simulink model "EV_BMS_SOC_Estimation_System"  (R2026a)
settings: Solver=ode4  StopTime=SCN.t_end  FixedStep=0.25
values from neighbouring files (symbols this model uses):
  BMS = struct('I_dis_cont', 20, 'I_chg_cont', 4,      'T_warn', 45, 'T_derate', 50, 'T_cutoff', 60,      'T_chg_min', 0, 'T_chg_low', 10, 'T_chg_max', 50,      'T_cold', -20, 'V_max', 4.20, 'V_min', 2.80, 'SOC_min', 0.05,      'enable', g('bms_enable', 1))    [ev_scenario.m]
  ET = struct()    [ET_Battery_Params.m]    (also in run_Extreme_Heat_Scenarios.m = apply_cooling(ET0, S{k,7}); run_Indian_Climate_Scenarios.m = apply_cooling(ET0, S{k,6}))
  PACK = struct('Ns', 20, 'Np', 14)    [ev_scenario.m]
  SCN = struct()    [ev_scenario.m]
  VEH = struct('name', 'Electric scooter', 'm', 195,              'Cd', 0.70, 'A', 0.85, 'Crr', 0.016, 'rho', 1.18, 'kr', 1.03,              'eta_drive', 0.85, 'eta_regen', 0.50, 'P_regen_max', 2e3,              'P_trac_max', 6e3, 'v_regen_min', 5)    [ev_scenario.m]
libraries: sl_discontinuities x1
settings Model: Creator=anand  LastModifiedBy=anand

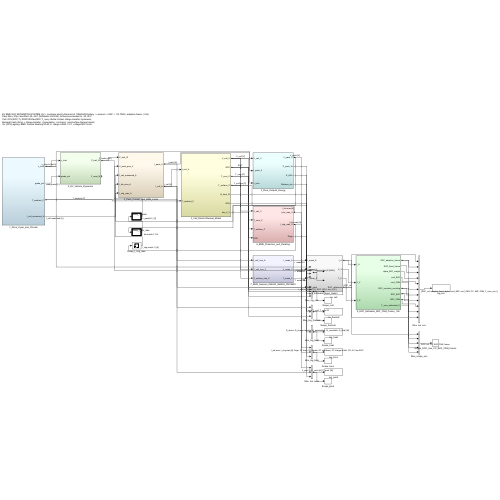
[thumbnail: Simulink's stored preview of the top-level diagram]
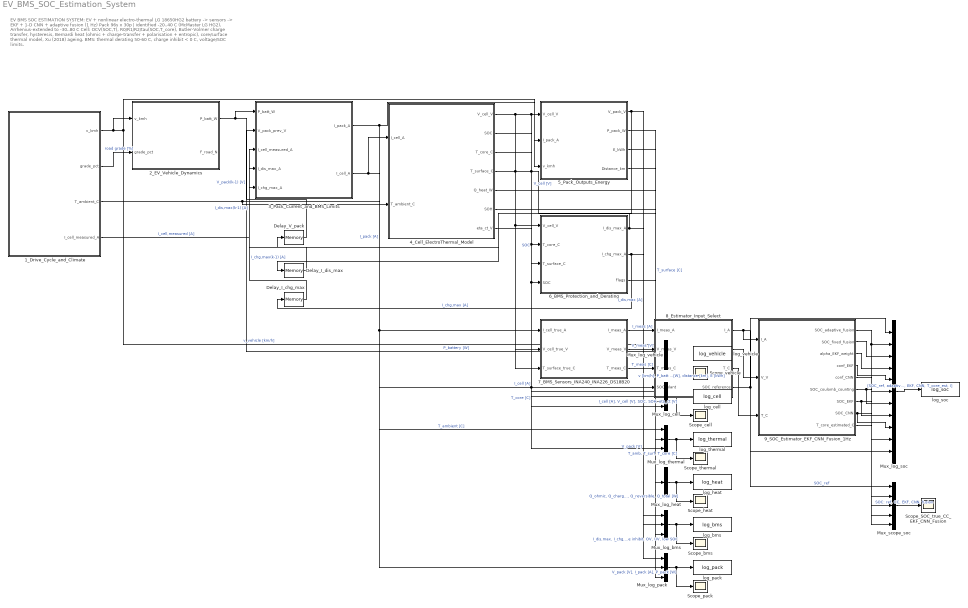
== system EV_BMS_SOC_Estimation_System ==
  note: EV BMS SOC ESTIMATION SYSTEM: EV + nonlinear electro-thermal LG 18650HG2 battery -> sensors -> EKF + 1-D CNN + adaptive fusion (1 Hz)
      | Pack 96s x 30p | identified -20..40 C (McMaster LG HG2), Arrhenius-extended to -30..80 C
      | Cell: OCV(SOC,T), R0/R1/R2/tau(SOC,T_core), Butler-Volmer charge transfer, hysteresis,
      | Bernardi heat (ohmic + charge-transfer + polarisation + entropic), core/surface thermal model,
      | Xu (2018) ageing. BMS: thermal derating 50-60 C, charge inhibit < 0 C, voltage/SOC limits.
  1_Drive_Cycle_and_Climate : Subsystem
  2_EV_Vehicle_Dynamics : Subsystem
  3_Pack_Current_and_BMS_Limits : Subsystem
  4_Cell_ElectroThermal_Model : Subsystem
  5_Pack_Outputs_Energy : Subsystem
  6_BMS_Protection_and_Derating : Subsystem
  7_BMS_Sensors_INA240_INA226_DS18B20 : Subsystem
  8_Estimator_Input_Select : Subsystem
  9_SOC_Estimator_EKF_CNN_Fusion_1Hz : Subsystem
  Delay_I_chg_max : Memory  InitialCondition=BMS.I_chg_cont*PACK.Np
  Delay_I_dis_max : Memory  InitialCondition=BMS.I_dis_cont*PACK.Np
  Delay_V_pack : Memory  InitialCondition=PACK.Ns*3.7
  Mux_log_bms : Mux  Inputs=3
  Mux_log_cell : Mux  Inputs=5
  Mux_log_heat : Mux  Inputs=1
  Mux_log_pack : Mux  Inputs=3
  Mux_log_soc : Mux  Inputs=11
  Mux_log_thermal : Mux  Inputs=3
  Mux_log_vehicle : Mux
  Mux_scope_soc : Mux  Inputs=5
  Scope_SOC_true_CC_EKF_CNN_Fusion : Scope
  Scope_bms : Scope
  Scope_cell : Scope
  Scope_heat : Scope
  Scope_pack : Scope
  Scope_thermal : Scope
  Scope_vehicle : Scope
  log_bms : ToWorkspace  VariableName=log_bms  SaveFormat=Timeseries  SampleTime=-1
  log_cell : ToWorkspace  VariableName=log_cell  SaveFormat=Timeseries  SampleTime=-1
  log_heat : ToWorkspace  VariableName=log_heat  SaveFormat=Timeseries  SampleTime=-1
  log_pack : ToWorkspace  VariableName=log_pack  SaveFormat=Timeseries  SampleTime=-1
  log_soc : ToWorkspace  VariableName=log_soc  SaveFormat=Timeseries  SampleTime=-1
  log_thermal : ToWorkspace  VariableName=log_thermal  SaveFormat=Timeseries  SampleTime=-1
  log_vehicle : ToWorkspace  VariableName=log_vehicle  SaveFormat=Timeseries  SampleTime=-1
  wires:
  1_Drive_Cycle_and_Climate/1(v_kmh) -> 5_Pack_Outputs_Energy/3(v_kmh), Mux_log_vehicle/1, 2_EV_Vehicle_Dynamics/1(v_kmh)  "v_vehicle [km/h]"
  1_Drive_Cycle_and_Climate/2(grade_pct) -> 2_EV_Vehicle_Dynamics/2(grade_pct)  "road grade [%]"
  1_Drive_Cycle_and_Climate/3(T_ambient_C) -> 4_Cell_ElectroThermal_Model/2(T_ambient_C), Mux_log_thermal/1  "T_ambient [C]"
  1_Drive_Cycle_and_Climate/4(I_cell_measured_A) -> 3_Pack_Current_and_BMS_Limits/3(I_cell_measured_A)  "I_cell,measured [A]"
  2_EV_Vehicle_Dynamics/1(P_batt_W) -> 3_Pack_Current_and_BMS_Limits/1(P_batt_W), Mux_log_vehicle/2  "P_battery [W]"
  Delay_V_pack/1 -> 3_Pack_Current_and_BMS_Limits/2(V_pack_prev_V)  "V_pack(k-1) [V]"
  Delay_I_dis_max/1 -> 3_Pack_Current_and_BMS_Limits/4(I_dis_max_A)  "I_dis,max(k-1) [A]"
  Delay_I_chg_max/1 -> 3_Pack_Current_and_BMS_Limits/5(I_chg_max_A)  "I_chg,max(k-1) [A]"
  3_Pack_Current_and_BMS_Limits/2(I_cell_A) -> Mux_log_cell/1, 7_BMS_Sensors_INA240_INA226_DS18B20/1(I_cell_true_A), 4_Cell_ElectroThermal_Model/1(I_cell_A)  "I_cell [A]"
  3_Pack_Current_and_BMS_Limits/1(I_pack_A) -> 5_Pack_Outputs_Energy/2(I_pack_A), Mux_log_pack/2  "I_pack [A]"
  4_Cell_ElectroThermal_Model/1(V_cell_V) -> 6_BMS_Protection_and_Derating/1(V_cell_V), 7_BMS_Sensors_INA240_INA226_DS18B20/2(V_cell_true_V), 5_Pack_Outputs_Energy/1(V_cell_V), Mux_log_cell/2  "V_cell [V]"
  5_Pack_Outputs_Energy/1(V_pack_V) -> Delay_V_pack/1, Mux_log_pack/1  "V_pack [V]"
  4_Cell_ElectroThermal_Model/3(T_core_C) -> 6_BMS_Protection_and_Derating/2(T_core_C), Mux_log_thermal/3  "T_core [C]"
  4_Cell_ElectroThermal_Model/4(T_surface_C) -> 6_BMS_Protection_and_Derating/3(T_surface_C), Mux_log_thermal/2, 7_BMS_Sensors_INA240_INA226_DS18B20/3(T_surface_true_C)  "T_surface [C]"
  4_Cell_ElectroThermal_Model/2(SOC) -> Mux_log_cell/3, 8_Estimator_Input_Select/4(SOC_plant), 6_BMS_Protection_and_Derating/4(SOC)  "SOC"
  6_BMS_Protection_and_Derating/1(I_dis_max_A) -> Delay_I_dis_max/1, Mux_log_bms/1  "I_dis,max [A]"
  6_BMS_Protection_and_Derating/2(I_chg_max_A) -> Delay_I_chg_max/1, Mux_log_bms/2  "I_chg,max [A]"
  5_Pack_Outputs_Energy/4(Distance_km) -> Mux_log_vehicle/3
  5_Pack_Outputs_Energy/3(E_kWh) -> Mux_log_vehicle/4
  Mux_log_vehicle/1 -> log_vehicle/1, Scope_vehicle/1  "v [km/h], P_batt [W], distance [km], E [kWh]"
  4_Cell_ElectroThermal_Model/6(SOH) -> Mux_log_cell/4
  4_Cell_ElectroThermal_Model/7(eta_ct_V) -> Mux_log_cell/5
  Mux_log_cell/1 -> log_cell/1, Scope_cell/1  "I_cell [A], V_cell [V], SOC, SOH, eta_ct [V]"
  Mux_log_thermal/1 -> log_thermal/1, Scope_thermal/1  "T_amb, T_surf, T_core [C]"
  4_Cell_ElectroThermal_Model/5(Q_heat_W) -> Mux_log_heat/1
  Mux_log_heat/1 -> log_heat/1, Scope_heat/1  "Q_ohmic, Q_charge-transfer, Q_polarisation, Q_reversible, Q_total [W]"
  6_BMS_Protection_and_Derating/3(Flags) -> Mux_log_bms/3
  Mux_log_bms/1 -> log_bms/1, Scope_bms/1  "I_dis,max, I_chg,max [A], flags: OT warn, OT derate, OT shutdown, UT charge inhibit, OV, UV, low SOC"
  5_Pack_Outputs_Energy/2(P_pack_W) -> Mux_log_pack/3
  Mux_log_pack/1 -> log_pack/1, Scope_pack/1  "V_pack [V], I_pack [A], P_pack [W]"
  7_BMS_Sensors_INA240_INA226_DS18B20/1(I_meas_A) -> 8_Estimator_Input_Select/1(I_meas_A)  "I_meas [A]"
  7_BMS_Sensors_INA240_INA226_DS18B20/2(V_meas_V) -> 8_Estimator_Input_Select/2(V_meas_V)  "V_meas [V]"
  7_BMS_Sensors_INA240_INA226_DS18B20/3(T_meas_C) -> 8_Estimator_Input_Select/3(T_meas_C)  "T_meas [C]"
  8_Estimator_Input_Select/1(I_A) -> 9_SOC_Estimator_EKF_CNN_Fusion_1Hz/1(I_A), Mux_log_soc/11
  8_Estimator_Input_Select/2(V_V) -> 9_SOC_Estimator_EKF_CNN_Fusion_1Hz/2(V_V)
  8_Estimator_Input_Select/3(T_C) -> 9_SOC_Estimator_EKF_CNN_Fusion_1Hz/3(T_C)
  8_Estimator_Input_Select/4(SOC_reference) -> Mux_log_soc/1, Mux_scope_soc/1  "SOC_ref"
  9_SOC_Estimator_EKF_CNN_Fusion_1Hz/1(SOC_adaptive_fusion) -> Mux_log_soc/2, Mux_scope_soc/5
  9_SOC_Estimator_EKF_CNN_Fusion_1Hz/2(SOC_fixed_fusion) -> Mux_log_soc/3
  9_SOC_Estimator_EKF_CNN_Fusion_1Hz/3(alpha_EKF_weight) -> Mux_log_soc/4
  9_SOC_Estimator_EKF_CNN_Fusion_1Hz/4(conf_EKF) -> Mux_log_soc/5
  9_SOC_Estimator_EKF_CNN_Fusion_1Hz/5(conf_CNN) -> Mux_log_soc/6
  9_SOC_Estimator_EKF_CNN_Fusion_1Hz/6(SOC_coulomb_counting) -> Mux_log_soc/7, Mux_scope_soc/2
  9_SOC_Estimator_EKF_CNN_Fusion_1Hz/7(SOC_EKF) -> Mux_log_soc/8, Mux_scope_soc/3
  9_SOC_Estimator_EKF_CNN_Fusion_1Hz/8(SOC_CNN) -> Mux_log_soc/9, Mux_scope_soc/4
  9_SOC_Estimator_EKF_CNN_Fusion_1Hz/9(T_core_estimated_C) -> Mux_log_soc/10
  Mux_log_soc/1 -> log_soc/1  "[SOC_ref, adaptive, fixed, alpha, conf_EKF, conf_CNN, CC, EKF, CNN, T_core_est, I]"
  Mux_scope_soc/1 -> Scope_SOC_true_CC_EKF_CNN_Fusion/1  "SOC: ref, CC, EKF, CNN, fusion"

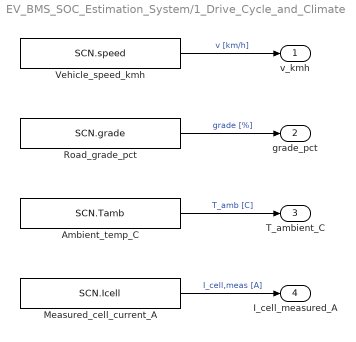
== system EV_BMS_SOC_Estimation_System/1_Drive_Cycle_and_Climate ==
  Ambient_temp_C : FromWorkspace  VariableName=SCN.Tamb  OutputAfterFinalValue=Holding final value
  Measured_cell_current_A : FromWorkspace  VariableName=SCN.Icell  Interpolate=off  OutputAfterFinalValue=Holding final value
  Road_grade_pct : FromWorkspace  VariableName=SCN.grade  OutputAfterFinalValue=Holding final value
  Vehicle_speed_kmh : FromWorkspace  VariableName=SCN.speed  OutputAfterFinalValue=Holding final value
  v_kmh : Outport
  grade_pct : Outport  Port=2
  T_ambient_C : Outport  Port=3
  I_cell_measured_A : Outport  Port=4
  wires:
  Vehicle_speed_kmh/1 -> v_kmh/1  "v [km/h]"
  Road_grade_pct/1 -> grade_pct/1  "grade [%]"
  Ambient_temp_C/1 -> T_ambient_C/1  "T_amb [C]"
  Measured_cell_current_A/1 -> I_cell_measured_A/1  "I_cell,meas [A]"

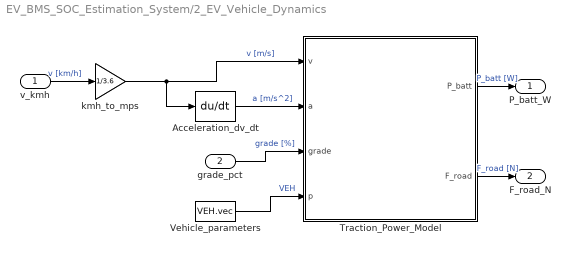
== system EV_BMS_SOC_Estimation_System/2_EV_Vehicle_Dynamics ==
  v_kmh : Inport
  grade_pct : Inport  Port=2
  Acceleration_dv_dt : Derivative
  Traction_Power_Model : MATLAB Function  TreatAsAtomicUnit=on
  Vehicle_parameters : Constant  Value=VEH.vec
  kmh_to_mps : Gain  Gain=1/3.6
  P_batt_W : Outport
  F_road_N : Outport  Port=2
  wires:
  v_kmh/1 -> kmh_to_mps/1  "v [km/h]"
  Traction_Power_Model/2(F_road) -> F_road_N/1  "F_road [N]"
  kmh_to_mps/1 -> Traction_Power_Model/1(v), Acceleration_dv_dt/1  "v [m/s]"
  Vehicle_parameters/1 -> Traction_Power_Model/4(p)  "VEH"
  Acceleration_dv_dt/1 -> Traction_Power_Model/2(a)  "a [m/s^2]"
  grade_pct/1 -> Traction_Power_Model/3(grade)  "grade [%]"
  Traction_Power_Model/1(P_batt) -> P_batt_W/1  "P_batt [W]"

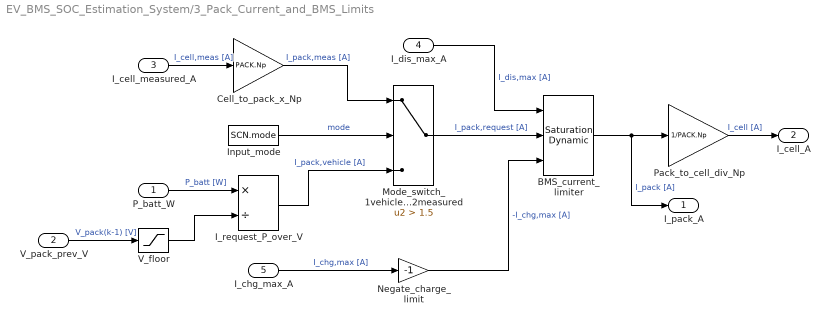
== system EV_BMS_SOC_Estimation_System/3_Pack_Current_and_BMS_Limits ==
  P_batt_W : Inport
  V_pack_prev_V : Inport  Port=2
  I_cell_measured_A : Inport  Port=3
  I_dis_max_A : Inport  Port=4
  I_chg_max_A : Inport  Port=5
  BMS_current_limiter : sl_discontinuities/Saturation Dynamic  OutMin=[]  OutMax=[]  OutDataTypeStr=Inherit: Same as second input  OutDataType=fixdt(1, 16)  OutScaling=2^-10  DoSatur=off
      settings: LibrarySourceBlock=|
      | simulink/Discontinuities/Saturation
      | Dynamic
  Cell_to_pack_x_Np : Gain  Gain=PACK.Np
  I_request_P_over_V : Product  Inputs=*/
  Input_mode : Constant  Value=SCN.mode
  Mode_switch_1vehicle_2measured : Switch  Criteria=u2 > Threshold  Threshold=1.5  SaturateOnIntegerOverflow=off  InputSameDT=off
  Negate_charge_limit : Gain  Gain=-1
  Pack_to_cell_div_Np : Gain  Gain=1/PACK.Np
  V_floor : Saturate  UpperLimit=inf  LowerLimit=1
  I_pack_A : Outport
  I_cell_A : Outport  Port=2
  wires:
  I_chg_max_A/1 -> Negate_charge_limit/1  "I_chg,max [A]"
  P_batt_W/1 -> I_request_P_over_V/1  "P_batt [W]"
  V_floor/1 -> I_request_P_over_V/2
  I_request_P_over_V/1 -> Mode_switch_1vehicle_2measured/3  "I_pack,vehicle [A]"
  Input_mode/1 -> Mode_switch_1vehicle_2measured/2  "mode"
  Cell_to_pack_x_Np/1 -> Mode_switch_1vehicle_2measured/1  "I_pack,meas [A]"
  I_cell_measured_A/1 -> Cell_to_pack_x_Np/1  "I_cell,meas [A]"
  V_pack_prev_V/1 -> V_floor/1  "V_pack(k-1) [V]"
  I_dis_max_A/1 -> BMS_current_limiter/1  "I_dis,max [A]"
  Mode_switch_1vehicle_2measured/1 -> BMS_current_limiter/2  "I_pack,request [A]"
  Negate_charge_limit/1 -> BMS_current_limiter/3  "-I_chg,max [A]"
  BMS_current_limiter/1 -> I_pack_A/1, Pack_to_cell_div_Np/1  "I_pack [A]"
  Pack_to_cell_div_Np/1 -> I_cell_A/1  "I_cell [A]"

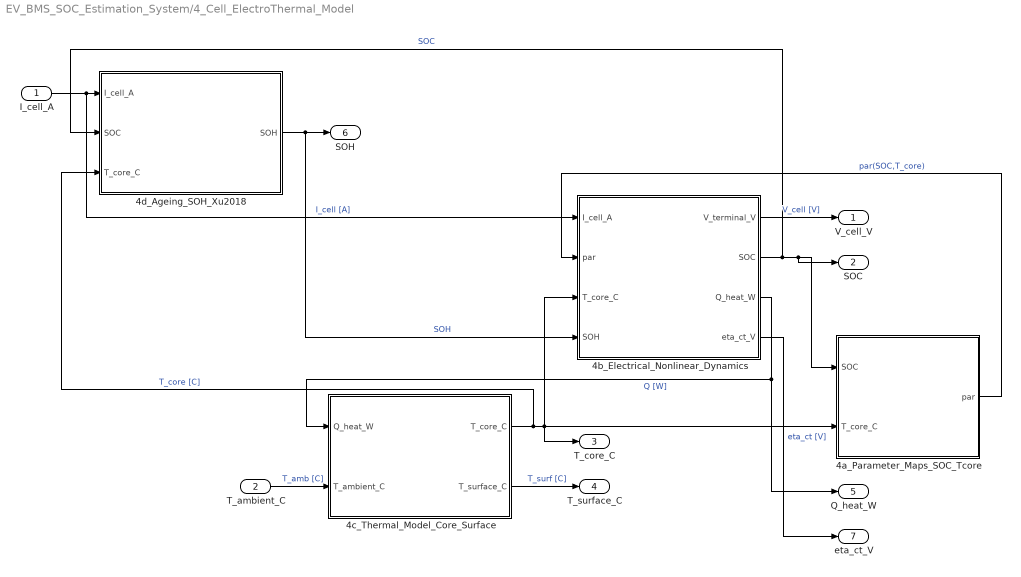
== system EV_BMS_SOC_Estimation_System/4_Cell_ElectroThermal_Model ==
  I_cell_A : Inport
  T_ambient_C : Inport  Port=2
  4a_Parameter_Maps_SOC_Tcore : Subsystem
  4b_Electrical_Nonlinear_Dynamics : Subsystem
  4c_Thermal_Model_Core_Surface : Subsystem
  4d_Ageing_SOH_Xu2018 : Subsystem
  V_cell_V : Outport
  SOC : Outport  Port=2
  T_core_C : Outport  Port=3
  T_surface_C : Outport  Port=4
  Q_heat_W : Outport  Port=5
  SOH : Outport  Port=6
  eta_ct_V : Outport  Port=7
  wires:
  4b_Electrical_Nonlinear_Dynamics/3(Q_heat_W) -> 4c_Thermal_Model_Core_Surface/1(Q_heat_W), Q_heat_W/1  "Q [W]"
  4b_Electrical_Nonlinear_Dynamics/1(V_terminal_V) -> V_cell_V/1  "V_cell [V]"
  T_ambient_C/1 -> 4c_Thermal_Model_Core_Surface/2(T_ambient_C)  "T_amb [C]"
  I_cell_A/1 -> 4b_Electrical_Nonlinear_Dynamics/1(I_cell_A), 4d_Ageing_SOH_Xu2018/1(I_cell_A)  "I_cell [A]"
  4d_Ageing_SOH_Xu2018/1(SOH) -> SOH/1, 4b_Electrical_Nonlinear_Dynamics/4(SOH)  "SOH"
  4c_Thermal_Model_Core_Surface/1(T_core_C) -> 4a_Parameter_Maps_SOC_Tcore/2(T_core_C), 4b_Electrical_Nonlinear_Dynamics/3(T_core_C), T_core_C/1, 4d_Ageing_SOH_Xu2018/3(T_core_C)  "T_core [C]"
  4c_Thermal_Model_Core_Surface/2(T_surface_C) -> T_surface_C/1  "T_surf [C]"
  4b_Electrical_Nonlinear_Dynamics/2(SOC) -> 4a_Parameter_Maps_SOC_Tcore/1(SOC), SOC/1, 4d_Ageing_SOH_Xu2018/2(SOC)  "SOC"
  4b_Electrical_Nonlinear_Dynamics/4(eta_ct_V) -> eta_ct_V/1  "eta_ct [V]"
  4a_Parameter_Maps_SOC_Tcore/1(par) -> 4b_Electrical_Nonlinear_Dynamics/2(par)  "par(SOC,T_core)"

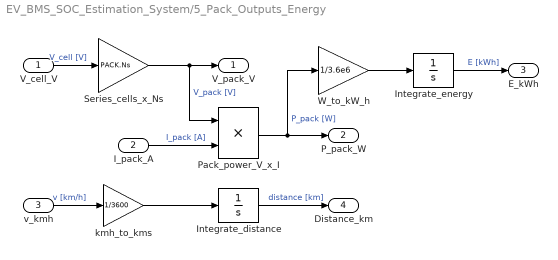
== system EV_BMS_SOC_Estimation_System/5_Pack_Outputs_Energy ==
  V_cell_V : Inport
  I_pack_A : Inport  Port=2
  v_kmh : Inport  Port=3
  Integrate_distance : Integrator
  Integrate_energy : Integrator
  Pack_power_V_x_I : Product
  Series_cells_x_Ns : Gain  Gain=PACK.Ns
  W_to_kW_h : Gain  Gain=1/3.6e6
  kmh_to_kms : Gain  Gain=1/3600
  V_pack_V : Outport
  P_pack_W : Outport  Port=2
  E_kWh : Outport  Port=3
  Distance_km : Outport  Port=4
  wires:
  Integrate_distance/1 -> Distance_km/1  "distance [km]"
  Pack_power_V_x_I/1 -> W_to_kW_h/1, P_pack_W/1  "P_pack [W]"
  Series_cells_x_Ns/1 -> V_pack_V/1, Pack_power_V_x_I/1  "V_pack [V]"
  v_kmh/1 -> kmh_to_kms/1  "v [km/h]"
  Integrate_energy/1 -> E_kWh/1  "E [kWh]"
  V_cell_V/1 -> Series_cells_x_Ns/1  "V_cell [V]"
  W_to_kW_h/1 -> Integrate_energy/1
  I_pack_A/1 -> Pack_power_V_x_I/2  "I_pack [A]"
  kmh_to_kms/1 -> Integrate_distance/1

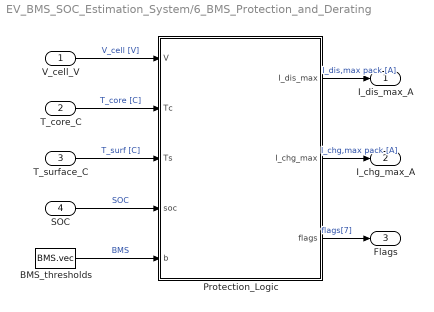
== system EV_BMS_SOC_Estimation_System/6_BMS_Protection_and_Derating ==
  V_cell_V : Inport
  T_core_C : Inport  Port=2
  T_surface_C : Inport  Port=3
  SOC : Inport  Port=4
  BMS_thresholds : Constant  Value=BMS.vec
  Protection_Logic : MATLAB Function  TreatAsAtomicUnit=on
  I_dis_max_A : Outport
  I_chg_max_A : Outport  Port=2
  Flags : Outport  Port=3
  wires:
  V_cell_V/1 -> Protection_Logic/1(V)  "V_cell [V]"
  Protection_Logic/2(I_chg_max) -> I_chg_max_A/1  "I_chg,max pack [A]"
  SOC/1 -> Protection_Logic/4(soc)  "SOC"
  T_core_C/1 -> Protection_Logic/2(Tc)  "T_core [C]"
  Protection_Logic/3(flags) -> Flags/1  "flags[7]"
  Protection_Logic/1(I_dis_max) -> I_dis_max_A/1  "I_dis,max pack [A]"
  BMS_thresholds/1 -> Protection_Logic/5(b)  "BMS"
  T_surface_C/1 -> Protection_Logic/3(Ts)  "T_surf [C]"

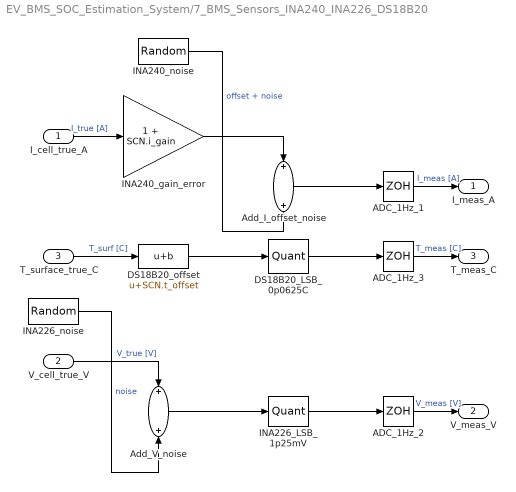
== system EV_BMS_SOC_Estimation_System/7_BMS_Sensors_INA240_INA226_DS18B20 ==
  I_cell_true_A : Inport
  V_cell_true_V : Inport  Port=2
  T_surface_true_C : Inport  Port=3
  ADC_1Hz_1 : ZeroOrderHold
  ADC_1Hz_2 : ZeroOrderHold
  ADC_1Hz_3 : ZeroOrderHold
  Add_I_offset_noise : Sum
  Add_V_noise : Sum
  DS18B20_LSB_0p0625C : Quantizer  QuantizationInterval=SCN.t_lsb
  DS18B20_offset : Bias  Bias=SCN.t_offset  SaturateOnIntegerOverflow=off
  INA226_LSB_1p25mV : Quantizer  QuantizationInterval=SCN.v_lsb
  INA226_noise : RandomNumber  Variance=SCN.v_noise^2  Seed=22  SampleTime=1
  INA240_gain_error : Gain  Gain=1 + SCN.i_gain
  INA240_noise : RandomNumber  Mean=SCN.i_offset  Variance=SCN.i_noise^2  Seed=11  SampleTime=1
  I_meas_A : Outport
  V_meas_V : Outport  Port=2
  T_meas_C : Outport  Port=3
  wires:
  Add_V_noise/1 -> INA226_LSB_1p25mV/1
  INA240_gain_error/1 -> Add_I_offset_noise/1
  INA240_noise/1 -> Add_I_offset_noise/2  "offset + noise"
  I_cell_true_A/1 -> INA240_gain_error/1  "I_true [A]"
  INA226_noise/1 -> Add_V_noise/2  "noise"
  Add_I_offset_noise/1 -> ADC_1Hz_1/1
  T_surface_true_C/1 -> DS18B20_offset/1  "T_surf [C]"
  V_cell_true_V/1 -> Add_V_noise/1  "V_true [V]"
  DS18B20_offset/1 -> DS18B20_LSB_0p0625C/1
  DS18B20_LSB_0p0625C/1 -> ADC_1Hz_3/1
  INA226_LSB_1p25mV/1 -> ADC_1Hz_2/1
  ADC_1Hz_1/1 -> I_meas_A/1  "I_meas [A]"
  ADC_1Hz_3/1 -> T_meas_C/1  "T_meas [C]"
  ADC_1Hz_2/1 -> V_meas_V/1  "V_meas [V]"

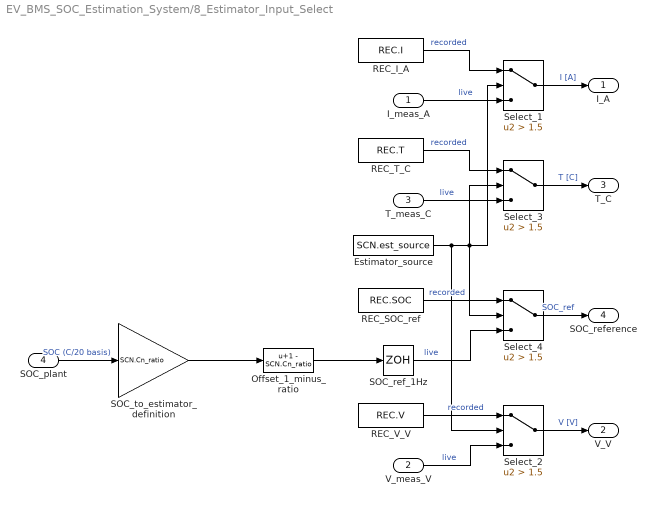
== system EV_BMS_SOC_Estimation_System/8_Estimator_Input_Select ==
  I_meas_A : Inport
  V_meas_V : Inport  Port=2
  T_meas_C : Inport  Port=3
  SOC_plant : Inport  Port=4
  Estimator_source : Constant  Value=SCN.est_source
  Offset_1_minus_ratio : Bias  Bias=1 - SCN.Cn_ratio  SaturateOnIntegerOverflow=off
  REC_I_A : FromWorkspace  VariableName=REC.I  SampleTime=1  Interpolate=off  OutputAfterFinalValue=Holding final value
  REC_SOC_ref : FromWorkspace  VariableName=REC.SOC  SampleTime=1  Interpolate=off  OutputAfterFinalValue=Holding final value
  REC_T_C : FromWorkspace  VariableName=REC.T  SampleTime=1  Interpolate=off  OutputAfterFinalValue=Holding final value
  REC_V_V : FromWorkspace  VariableName=REC.V  SampleTime=1  Interpolate=off  OutputAfterFinalValue=Holding final value
  SOC_ref_1Hz : ZeroOrderHold
  SOC_to_estimator_definition : Gain  Gain=SCN.Cn_ratio
  Select_{1..4} (4 alike) : Switch  Criteria=u2 > Threshold  Threshold=1.5  SaturateOnIntegerOverflow=off  InputSameDT=off
  I_A : Outport
  V_V : Outport  Port=2
  T_C : Outport  Port=3
  SOC_reference : Outport  Port=4
  wires:
  SOC_to_estimator_definition/1 -> Offset_1_minus_ratio/1
  SOC_plant/1 -> SOC_to_estimator_definition/1  "SOC (C/20 basis)"
  Offset_1_minus_ratio/1 -> SOC_ref_1Hz/1
  REC_T_C/1 -> Select_3/1  "recorded"
  Estimator_source/1 -> Select_1/2, Select_3/2, Select_4/2, Select_2/2
  REC_I_A/1 -> Select_1/1  "recorded"
  T_meas_C/1 -> Select_3/3  "live"
  I_meas_A/1 -> Select_1/3  "live"
  Select_1/1 -> I_A/1  "I [A]"
  REC_SOC_ref/1 -> Select_4/1  "recorded"
  Select_2/1 -> V_V/1  "V [V]"
  SOC_ref_1Hz/1 -> Select_4/3  "live"
  REC_V_V/1 -> Select_2/1  "recorded"
  V_meas_V/1 -> Select_2/3  "live"
  Select_3/1 -> T_C/1  "T [C]"
  Select_4/1 -> SOC_reference/1  "SOC_ref"

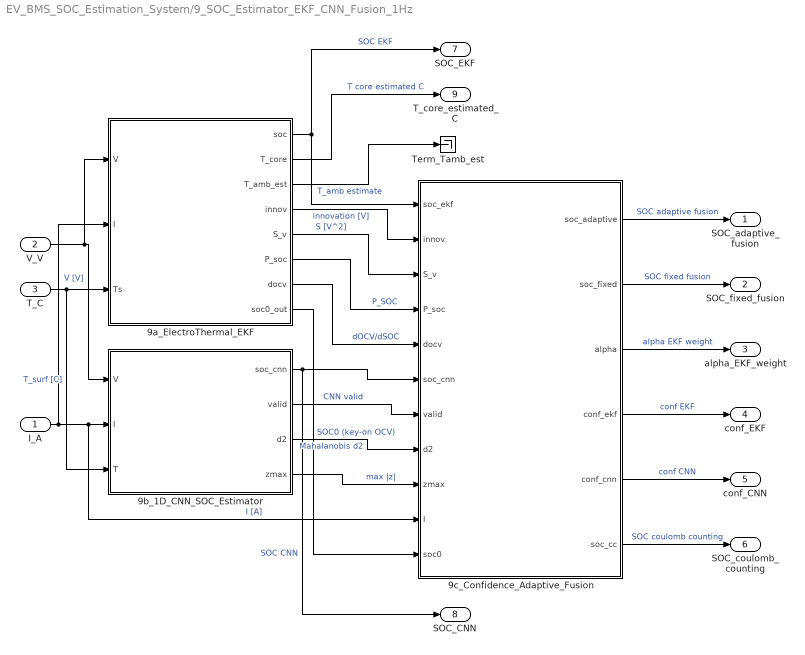
== system EV_BMS_SOC_Estimation_System/9_SOC_Estimator_EKF_CNN_Fusion_1Hz ==
  I_A : Inport
  V_V : Inport  Port=2
  T_C : Inport  Port=3
  9a_ElectroThermal_EKF : MATLAB Function  TreatAsAtomicUnit=on
  9b_1D_CNN_SOC_Estimator : MATLAB Function  TreatAsAtomicUnit=on
  9c_Confidence_Adaptive_Fusion : MATLAB Function  TreatAsAtomicUnit=on
  Term_Tamb_est : Terminator
  SOC_adaptive_fusion : Outport
  SOC_fixed_fusion : Outport  Port=2
  alpha_EKF_weight : Outport  Port=3
  conf_EKF : Outport  Port=4
  conf_CNN : Outport  Port=5
  SOC_coulomb_counting : Outport  Port=6
  SOC_EKF : Outport  Port=7
  SOC_CNN : Outport  Port=8
  T_core_estimated_C : Outport  Port=9
  wires:
  9a_ElectroThermal_EKF/1(soc) -> 9c_Confidence_Adaptive_Fusion/1(soc_ekf), SOC_EKF/1  "SOC EKF"
  9a_ElectroThermal_EKF/5(S_v) -> 9c_Confidence_Adaptive_Fusion/3(S_v)  "S [V^2]"
  9a_ElectroThermal_EKF/3(T_amb_est) -> Term_Tamb_est/1  "T_amb estimate"
  V_V/1 -> 9a_ElectroThermal_EKF/1(V), 9b_1D_CNN_SOC_Estimator/1(V)  "V [V]"
  9a_ElectroThermal_EKF/4(innov) -> 9c_Confidence_Adaptive_Fusion/2(innov)  "innovation [V]"
  9a_ElectroThermal_EKF/2(T_core) -> T_core_estimated_C/1  "T core estimated C"
  I_A/1 -> 9b_1D_CNN_SOC_Estimator/2(I), 9c_Confidence_Adaptive_Fusion/10(I), 9a_ElectroThermal_EKF/2(I)  "I [A]"
  T_C/1 -> 9b_1D_CNN_SOC_Estimator/3(T), 9a_ElectroThermal_EKF/3(Ts)  "T_surf [C]"
  9a_ElectroThermal_EKF/6(P_soc) -> 9c_Confidence_Adaptive_Fusion/4(P_soc)  "P_SOC"
  9a_ElectroThermal_EKF/7(docv) -> 9c_Confidence_Adaptive_Fusion/5(docv)  "dOCV/dSOC"
  9a_ElectroThermal_EKF/8(soc0_out) -> 9c_Confidence_Adaptive_Fusion/11(soc0)  "SOC0 (key-on OCV)"
  9b_1D_CNN_SOC_Estimator/1(soc_cnn) -> 9c_Confidence_Adaptive_Fusion/6(soc_cnn), SOC_CNN/1  "SOC CNN"
  9b_1D_CNN_SOC_Estimator/2(valid) -> 9c_Confidence_Adaptive_Fusion/7(valid)  "CNN valid"
  9b_1D_CNN_SOC_Estimator/3(d2) -> 9c_Confidence_Adaptive_Fusion/8(d2)  "Mahalanobis d2"
  9b_1D_CNN_SOC_Estimator/4(zmax) -> 9c_Confidence_Adaptive_Fusion/9(zmax)  "max |z|"
  9c_Confidence_Adaptive_Fusion/1(soc_adaptive) -> SOC_adaptive_fusion/1  "SOC adaptive fusion"
  9c_Confidence_Adaptive_Fusion/2(soc_fixed) -> SOC_fixed_fusion/1  "SOC fixed fusion"
  9c_Confidence_Adaptive_Fusion/3(alpha) -> alpha_EKF_weight/1  "alpha EKF weight"
  9c_Confidence_Adaptive_Fusion/4(conf_ekf) -> conf_EKF/1  "conf EKF"
  9c_Confidence_Adaptive_Fusion/5(conf_cnn) -> conf_CNN/1  "conf CNN"
  9c_Confidence_Adaptive_Fusion/6(soc_cc) -> SOC_coulomb_counting/1  "SOC coulomb counting"

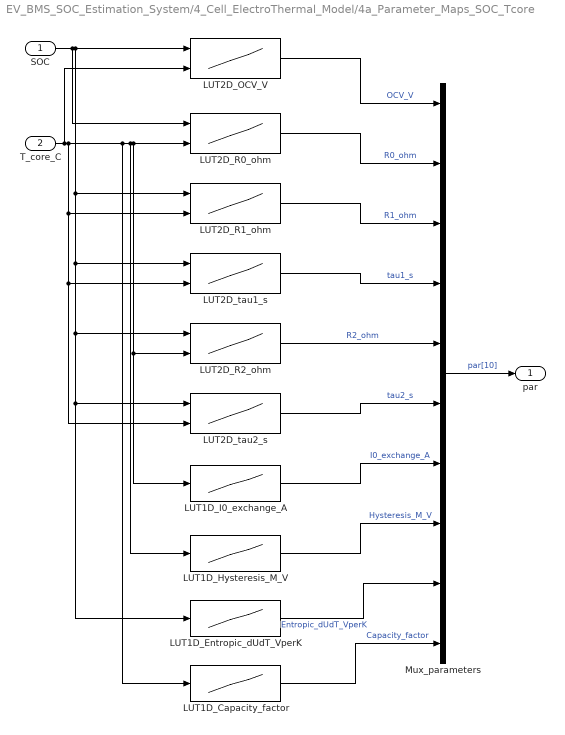
== system EV_BMS_SOC_Estimation_System/4_Cell_ElectroThermal_Model/4a_Parameter_Maps_SOC_Tcore ==
  SOC : Inport
  T_core_C : Inport  Port=2
  LUT1D_Capacity_factor : Lookup_n-D  NumberOfTableDimensions=1  BreakpointsForDimension1=ET.T_bp  Table=ET.cap_factor  ExtrapMethod=Clip  InternalRulePriority=Speed  RndMeth=Simplest
  LUT1D_Entropic_dUdT_VperK : Lookup_n-D  NumberOfTableDimensions=1  BreakpointsForDimension1=ET.soc_bp  Table=ET.dUdT  ExtrapMethod=Clip  InternalRulePriority=Speed  RndMeth=Simplest
  LUT1D_Hysteresis_M_V : Lookup_n-D  NumberOfTableDimensions=1  BreakpointsForDimension1=ET.T_bp  Table=ET.hyst_M  ExtrapMethod=Clip  InternalRulePriority=Speed  RndMeth=Simplest
  LUT1D_I0_exchange_A : Lookup_n-D  NumberOfTableDimensions=1  BreakpointsForDimension1=ET.T_bp  Table=ET.I0  ExtrapMethod=Clip  InternalRulePriority=Speed  RndMeth=Simplest
  LUT2D_OCV_V : Lookup_n-D  BreakpointsForDimension1=ET.soc_bp  BreakpointsForDimension2=ET.T_bp  Table=ET.OCV  ExtrapMethod=Clip  InternalRulePriority=Speed  RndMeth=Simplest
      settings: InputPortMap=u0,u1
  LUT2D_R0_ohm : Lookup_n-D  BreakpointsForDimension1=ET.soc_bp  BreakpointsForDimension2=ET.T_bp  Table=ET.R0  ExtrapMethod=Clip  InternalRulePriority=Speed  RndMeth=Simplest
      settings: InputPortMap=u0,u1
  LUT2D_R1_ohm : Lookup_n-D  BreakpointsForDimension1=ET.soc_bp  BreakpointsForDimension2=ET.T_bp  Table=ET.R1  ExtrapMethod=Clip  InternalRulePriority=Speed  RndMeth=Simplest
      settings: InputPortMap=u0,u1
  LUT2D_R2_ohm : Lookup_n-D  BreakpointsForDimension1=ET.soc_bp  BreakpointsForDimension2=ET.T_bp  Table=ET.R2  ExtrapMethod=Clip  InternalRulePriority=Speed  RndMeth=Simplest
      settings: InputPortMap=u0,u1
  LUT2D_tau1_s : Lookup_n-D  BreakpointsForDimension1=ET.soc_bp  BreakpointsForDimension2=ET.T_bp  Table=ET.tau1  ExtrapMethod=Clip  InternalRulePriority=Speed  RndMeth=Simplest
      settings: InputPortMap=u0,u1
  LUT2D_tau2_s : Lookup_n-D  BreakpointsForDimension1=ET.soc_bp  BreakpointsForDimension2=ET.T_bp  Table=ET.tau2  ExtrapMethod=Clip  InternalRulePriority=Speed  RndMeth=Simplest
      settings: InputPortMap=u0,u1
  Mux_parameters : Mux  Inputs=10
  par : Outport
  wires:
  T_core_C/1 -> LUT2D_tau1_s/2, LUT2D_tau2_s/2, LUT2D_R1_ohm/2, LUT1D_I0_exchange_A/1, LUT2D_R2_ohm/2, LUT2D_R0_ohm/2, LUT1D_Hysteresis_M_V/1, LUT1D_Capacity_factor/1, LUT2D_OCV_V/2
  SOC/1 -> LUT2D_tau2_s/1, LUT1D_Entropic_dUdT_VperK/1, LUT2D_R2_ohm/1, LUT2D_tau1_s/1, LUT2D_R1_ohm/1, LUT2D_OCV_V/1, LUT2D_R0_ohm/1
  LUT2D_R0_ohm/1 -> Mux_parameters/2  "R0_ohm"
  LUT2D_tau1_s/1 -> Mux_parameters/4  "tau1_s"
  LUT2D_OCV_V/1 -> Mux_parameters/1  "OCV_V"
  LUT2D_R1_ohm/1 -> Mux_parameters/3  "R1_ohm"
  LUT2D_tau2_s/1 -> Mux_parameters/6  "tau2_s"
  LUT1D_I0_exchange_A/1 -> Mux_parameters/7  "I0_exchange_A"
  LUT2D_R2_ohm/1 -> Mux_parameters/5  "R2_ohm"
  LUT1D_Hysteresis_M_V/1 -> Mux_parameters/8  "Hysteresis_M_V"
  LUT1D_Entropic_dUdT_VperK/1 -> Mux_parameters/9  "Entropic_dUdT_VperK"
  LUT1D_Capacity_factor/1 -> Mux_parameters/10  "Capacity_factor"
  Mux_parameters/1 -> par/1  "par[10]"

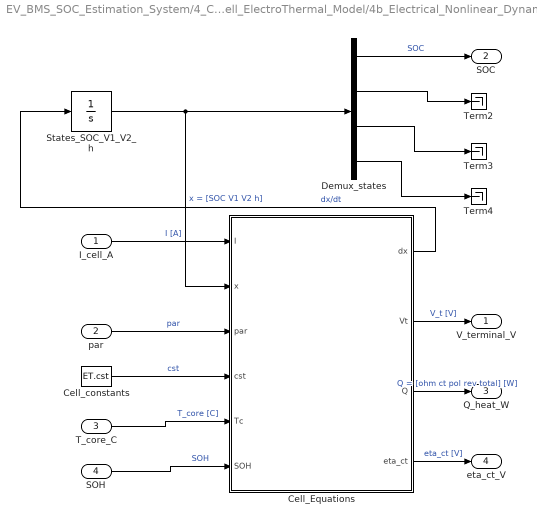
== system EV_BMS_SOC_Estimation_System/4_Cell_ElectroThermal_Model/4b_Electrical_Nonlinear_Dynamics ==
  I_cell_A : Inport
  par : Inport  Port=2
  T_core_C : Inport  Port=3
  SOH : Inport  Port=4
  Cell_Equations : MATLAB Function  TreatAsAtomicUnit=on
  Cell_constants : Constant  Value=ET.cst
  Demux_states : Demux
  States_SOC_V1_V2_h : Integrator  InitialCondition=[SCN.soc0; 0; 0; 0]
  Term2 : Terminator
  Term3 : Terminator
  Term4 : Terminator
  V_terminal_V : Outport
  SOC : Outport  Port=2
  Q_heat_W : Outport  Port=3
  eta_ct_V : Outport  Port=4
  wires:
  Cell_Equations/4(eta_ct) -> eta_ct_V/1  "eta_ct [V]"
  States_SOC_V1_V2_h/1 -> Cell_Equations/2(x), Demux_states/1  "x = [SOC V1 V2 h]"
  I_cell_A/1 -> Cell_Equations/1(I)  "I [A]"
  Demux_states/2 -> Term2/1
  T_core_C/1 -> Cell_Equations/5(Tc)  "T_core [C]"
  par/1 -> Cell_Equations/3(par)  "par"
  SOH/1 -> Cell_Equations/6(SOH)  "SOH"
  Cell_constants/1 -> Cell_Equations/4(cst)  "cst"
  Demux_states/1 -> SOC/1  "SOC"
  Demux_states/3 -> Term3/1
  Demux_states/4 -> Term4/1
  Cell_Equations/1(dx) -> States_SOC_V1_V2_h/1  "dx/dt"
  Cell_Equations/2(Vt) -> V_terminal_V/1  "V_t [V]"
  Cell_Equations/3(Q) -> Q_heat_W/1  "Q = [ohm ct pol rev total] [W]"

== system EV_BMS_SOC_Estimation_System/4_Cell_ElectroThermal_Model/4c_Thermal_Model_Core_Surface ==
  Q_heat_W : Inport
  T_ambient_C : Inport  Port=2
  Demux_T : Demux  Outputs=2
  Mux_Q_Tamb : Mux  Inputs=2
  Select_Q_total : Selector  InputPortWidth=5  IndexOptions=Index vector (dialog)  Indices=5  OutputSizes=1
  Two_state_thermal_Cc_Cs_Rc_Ru : StateSpace  A=ET.A_th  B=ET.B_th  C=eye(2)  D=zeros(2)  InitialCondition=[SCN.T0; SCN.T0]
  T_core_C : Outport
  T_surface_C : Outport  Port=2
  wires:
  Two_state_thermal_Cc_Cs_Rc_Ru/1 -> Demux_T/1  "[T_core; T_surf]"
  Mux_Q_Tamb/1 -> Two_state_thermal_Cc_Cs_Rc_Ru/1  "[Q; T_amb]"
  Select_Q_total/1 -> Mux_Q_Tamb/1  "Q_total [W]"
  Q_heat_W/1 -> Select_Q_total/1  "Q vector"
  T_ambient_C/1 -> Mux_Q_Tamb/2  "T_amb [C]"
  Demux_T/1 -> T_core_C/1  "T_core [C]"
  Demux_T/2 -> T_surface_C/1  "T_surf [C]"

== system EV_BMS_SOC_Estimation_System/4_Cell_ElectroThermal_Model/4d_Ageing_SOH_Xu2018 ==
  I_cell_A : Inport
  SOC : Inport  Port=2
  T_core_C : Inport  Port=3
  Ageing_coefficients : Constant  Value=[ET.xu(:); SCN.SOH0; ET.Cn_Ah]
  Degradation_fd : Integrator
  Xu_Stress_Model : MATLAB Function  TreatAsAtomicUnit=on
  SOH : Outport
  wires:
  Degradation_fd/1 -> Xu_Stress_Model/4(fd)  "f_d"
  Xu_Stress_Model/1(dfd) -> Degradation_fd/1  "df_d/dt"
  T_core_C/1 -> Xu_Stress_Model/3(Tc)  "T_core [C]"
  I_cell_A/1 -> Xu_Stress_Model/1(I)  "I [A]"
  Ageing_coefficients/1 -> Xu_Stress_Model/5(xu)  "xu"
  SOC/1 -> Xu_Stress_Model/2(soc)  "SOC"
  Xu_Stress_Model/2(SOH) -> SOH/1  "SOH"

== matlab function EV_BMS_SOC_Estimation_System/9_SOC_Estimator_EKF_CNN_Fusion_1Hz/9c_Confidence_Adaptive_Fusion ==
  data: soc_ekf input; soc_adaptive output; innov input; S_v input; P_soc input; docv input; soc_cnn input; valid input; d2 input; zmax input; I input; soc0 input; soc_fixed output; alpha output; conf_ekf output; conf_cnn output; soc_cc output
function [soc_adaptive, soc_fixed, alpha, conf_ekf, conf_cnn, soc_cc] = Adaptive_Fusion(soc_ekf, innov, S_v, P_soc, docv, soc_cnn, valid, d2, zmax, I, soc0)
%#codegen
% Confidence-based adaptive fusion, 1 Hz:
%   alpha = rho*c_ekf^beta / (rho*c_ekf^beta + c_cnn^beta), slew-limited
%   SOC = alpha*SOC_ekf + (1-alpha)*SOC_cnn
% c_ekf: innovation consistency, covariance, observability (|dOCV/dSOC|)
% c_cnn: prediction stability, agreement with Coulomb-counted dSOC, in-distribution
F = coder.load('SOC_Estimator_Params.mat');
persistent a cc hist cch n
if isempty(n)
    a = 1; cc = soc0; hist = zeros(10,1); cch = zeros(10,1); n = 0;
end
eps0 = F.fu_eps;
% Coulomb counting (baseline, and the physics check for the CNN), from the EKF key-on SOC
soc_cc = min(max(cc, 0), 1);
% ---- EKF confidence ----
zi = innov/sqrt(max(S_v, 1e-12));
f_in = exp(-0.5*(zi/F.fu_innov_k)^2);
f_cov = exp(-P_soc/F.fu_P_ref);
f_obs = min(max(abs(docv)/F.fu_g_ref, 0), 1);
conf_ekf = wgeom([f_in f_cov f_obs], [1 1 1.5], eps0);
% ---- CNN confidence ----
conf_cnn = 0;
if valid > 0
    n = n + 1;
    hist = [hist(2:end); soc_cnn]; cch = [cch(2:end); soc_cc];
    m = min(n, 10);
    if m >= 2
        seg = hist(11-m:10);
        f_st = exp(-std(seg, 1)/F.fu_stab_ref);
        f_ph = exp(-abs((hist(10) - hist(11-m)) - (cch(10) - cch(11-m)))/F.fu_phys_ref);
    else
        f_st = 1; f_ph = 1;
    end
    f_ood = 1/(1 + (max(d2,0)/F.ood_ref_d2)^3) / (1 + (max(zmax,0)/F.ood_ref_z)^3);
    conf_cnn = wgeom([f_st f_ph f_ood], [1 1 1.5], eps0);
    cp = max(conf_ekf, eps0); cm = max(conf_cnn, eps0);
    wp = F.fu_rho*cp^F.fu_beta; wm = cm^F.fu_beta;
    alpha_raw = wp/(wp + wm);
else
    alpha_raw = 1;
end
a = a + min(max(alpha_raw - a, -F.fu_slew), F.fu_slew);
alpha = a;
if valid > 0
    soc_adaptive = min(max(alpha*soc_ekf + (1 - alpha)*soc_cnn, 0), 1);
    soc_fixed = min(max(0.5*soc_ekf + 0.5*soc_cnn, 0), 1);
else
    soc_adaptive = soc_ekf; soc_fixed = soc_ekf;
end
% advance Coulomb counter
if I >= 0, eta = 1; else, eta = F.cc_eta_chg; end
cc = cc - eta*I/(3600*F.Cn);
end

function g = wgeom(t, wt, e)
g = exp(sum(wt .* log(max(t, e)))/sum(wt));
end

== matlab function EV_BMS_SOC_Estimation_System/4_Cell_ElectroThermal_Model/4b_Electrical_Nonlinear_Dynamics/Cell_Equations ==
  data: I input; dx output; x input; par input; cst input; Tc input; SOH input; Vt output; Q output; eta_ct output
function [dx, Vt, Q, eta_ct] = Cell_Equations(I, x, par, cst, Tc, SOH)
%#codegen
% Nonlinear electro-thermal cell, I > 0 discharge. x = [SOC; V1; V2; h]
% par = [OCV R0 R1 tau1 R2 tau2 I0 M dUdT capf] at (SOC, T_core)
% cst = [Cn_Ah eta_chg gamma k_R]
soc = x(1); v1 = x(2); v2 = x(3); h = x(4);
Cn = cst(1); eta_chg = cst(2); gam = cst(3); kR = cst(4);
SOH = max(SOH, 0.5);
g = 1 + kR*(1 - SOH);                   % resistance growth with ageing
OCV = par(1); R0 = g*par(2); R1 = g*par(3); tau1 = max(par(4), 1e-3);
R2 = g*par(5); tau2 = max(par(6), 1e-3); I0 = max(par(7), 1e-3)/g;
M = par(8); dUdT = par(9); capf = par(10);
TK = Tc + 273.15;
% Butler-Volmer charge-transfer overpotential (theoretical Tafel slope)
eta_ct = 2*8.314462618*TK/96485.33212*asinh(I/(2*I0));
if I >= 0
    eta = 1;
else
    eta = eta_chg;
end
dsoc = -eta*I/(3600*Cn*capf*SOH);
dv1 = (R1*I - v1)/tau1;                 % fast polarisation
dv2 = (R2*I - v2)/tau2;                 % diffusion polarisation
dh  = -gam*abs(dsoc)*(h + sign(I));     % one-state hysteresis (Plett)
dx = [dsoc; dv1; dv2; dh];
Vt = OCV + M*h - I*R0 - eta_ct - v1 - v2;
% Bernardi heat generation [W]: Q = I*(OCV - Vt) - I*T*dU/dT, split by source
Q_ohm = I^2*R0;
Q_ct  = I*eta_ct;
Q_pol = I*(v1 + v2);                   % Bernardi: current x polarisation
Q_rev = -I*TK*dUdT;
Q = [Q_ohm; Q_ct; Q_pol; Q_rev; Q_ohm + Q_ct + Q_pol + Q_rev];
end

== matlab function EV_BMS_SOC_Estimation_System/2_EV_Vehicle_Dynamics/Traction_Power_Model ==
  data: v input; P_batt output; a input; grade input; p input; F_road output
function [P_batt, F_road] = Traction_Power_Model(v, a, grade, p)
%#codegen
% Longitudinal EV dynamics. v [m/s], a [m/s^2], grade [%], p = VEH.vec
% p = [m Cd A Crr rho kr eta_drive eta_regen P_regen_max P_aux v_regen_min P_trac_max]
m = p(1); Cd = p(2); A = p(3); Crr = p(4); rho = p(5); kr = p(6);
eta_d = p(7); eta_r = p(8); Preg_max = p(9); P_aux = p(10);
v_reg_min = p(11)/3.6; Ptr_max = p(12);
th = atan(grade/100);
F_aero  = 0.5*rho*Cd*A*v^2;
F_roll  = m*9.81*Crr*cos(th)*(v > 0.1);
F_grade = m*9.81*sin(th);
F_inert = kr*m*a;
F_road = F_aero + F_roll + F_grade + F_inert;
P_wheel = F_road*v;
if P_wheel >= 0
    P_mot = min(P_wheel, Ptr_max)/eta_d;          % traction
elseif v > v_reg_min
    P_mot = max(P_wheel*eta_r, -Preg_max);        % regenerative braking
else
    P_mot = 0;                                    % friction brakes only
end
P_batt = P_mot + P_aux;
end

== matlab function EV_BMS_SOC_Estimation_System/4_Cell_ElectroThermal_Model/4d_Ageing_SOH_Xu2018/Xu_Stress_Model ==
  data: I input; dfd output; soc input; Tc input; fd input; xu input; SOH output
function [dfd, SOH] = Xu_Stress_Model(I, soc, Tc, fd, xu)
%#codegen
% Semi-empirical degradation, Xu et al., IEEE Trans. Smart Grid 9(2), 2018.
% xu = [a_sei b_sei k_d1 k_d2 k_d3 k_s s_ref k_T T_ref k_t T_min DoD_ref SOH0 Cn]
a = xu(1); b = xu(2); kd1 = xu(3); kd2 = xu(4); kd3 = xu(5);
ks = xu(6); sref = xu(7); kT = xu(8); Tref = xu(9) + 273.15; kt = xu(10);
Tmin = xu(11); DoD = xu(12); SOH0 = xu(13); Cn = xu(14);
T = max(Tc, Tmin) + 273.15;             % law valid above 15 C (paper)
S_T = exp(kT*(T - Tref)*Tref/T);
S_s = exp(ks*(soc - sref));
S_d = 1/(kd1*DoD^kd2 + kd3);            % stress of one cycle of depth DoD
cyc_rate = abs(I)/(2*3600*Cn)/DoD;      % cycles of depth DoD per second
dfd = (kt + cyc_rate*S_d)*S_s*S_T;      % calendar + cycling
L = 1 - a*exp(-b*fd) - (1 - a)*exp(-fd);
SOH = SOH0*(1 - L);
end

== matlab function EV_BMS_SOC_Estimation_System/6_BMS_Protection_and_Derating/Protection_Logic ==
  data: V input; I_dis_max output; Tc input; Ts input; soc input; b input; I_chg_max output; flags output
function [I_dis_max, I_chg_max, flags] = Protection_Logic(V, Tc, Ts, soc, b)
%#codegen
% b = [I_dis I_chg T_warn T_derate T_cutoff T_chg_min T_chg_low T_chg_max
%      T_cold V_max V_min SOC_min Np enable]
Idis = b(1); Ichg = b(2); Tw = b(3); Td = b(4); Tcut = b(5);
Tcmin = b(6); Tclow = b(7); Tcmax = b(8); Tcold = b(9);
Vmax = b(10); Vmin = b(11); SOCmin = b(12); Np = b(13); en = b(14);
T = max(Tc, Ts);                        % hottest node (core estimate)
% discharge derating: full below T_derate, linear to zero at T_cutoff
fd = min(max((Tcut - T)/(Tcut - Td), 0), 1);
if T < Tcold, fd = 0.25*fd; end         % extreme cold: limit power
% charge window: none below T_chg_min (Li plating), half up to T_chg_low
if T < Tcmin
    fc = 0;
elseif T < Tclow
    fc = 0.5;
else
    fc = min(max((Tcmax - T)/(Tcmax - Td + 1e-6), 0), 1);
end
OV = double(V >= Vmax); UV = double(V <= Vmin); LS = double(soc <= SOCmin);
if OV > 0, fc = 0; end
if UV > 0 || LS > 0, fd = 0; end
flags = [double(T >= Tw); double(T >= Td); double(T >= Tcut); ...
         double(T < Tcmin); OV; UV; LS];
if en > 0
    I_dis_max = fd*Idis*Np; I_chg_max = fc*Ichg*Np;
else
    I_dis_max = 1e6; I_chg_max = 1e6;    % protection disabled (validation runs)
end
end

== matlab function EV_BMS_SOC_Estimation_System/9_SOC_Estimator_EKF_CNN_Fusion_1Hz/9a_ElectroThermal_EKF ==
  data: V input; soc output; I input; Ts input; T_core output; T_amb_est output; innov output; S_v output; P_soc output; docv output; soc0_out output
function [soc, T_core, T_amb_est, innov, S_v, P_soc, docv, soc0_out] = ElectroThermal_EKF(V, I, Ts)
%#codegen
% Electro-thermal EKF, 1 Hz. x = [SOC V1 V2 T_core T_surf T_amb], z = [V; T_surf].
% Parameters scheduled on the estimated core temperature (falls back to the
% measured surface temperature after a thermal event the model cannot follow).
E = coder.load('SOC_Estimator_Params.mat');   % compile-time constants
persistent x P h w s0 init
if isempty(init)
    s0 = soc_from_v(E, V, Ts);                     % key-on SOC from the rested OCV
    x = [s0; 0; 0; Ts; Ts; Ts]; P = diag(E.ekf_P0); h = 0; w = 1; init = 1;
end
dt = 1;
soc0_out = s0;
% ---------------- measurement update ----------------
Tel = w*x(4) + (1-w)*Ts;
[v, ds, ~] = lut2(E, x(1), Tel);
M = interp1(E.T_bp, E.hyst_M_T, min(max(Tel,E.T_bp(1)),E.T_bp(end)));
I0 = interp1(E.T_bp, E.I0_T, min(max(Tel,E.T_bp(1)),E.T_bp(end)));
eta_ct = 2*8.314462618*(Tel + 273.15)/96485.33212*asinh(I/(2*I0));   % Butler-Volmer
yv = v(1) + M*h - I*v(2) - eta_ct - x(2) - x(3);
H = zeros(2,6); H(1,1) = ds(1) - I*ds(2); H(1,2) = -1; H(1,3) = -1; H(2,5) = 1;
Rm = diag([E.ekf_Rv, E.ekf_Rt]);
e = [V; Ts] - [yv; x(5)];
st = P(5,5) + Rm(2,2);
if e(2)^2/st > E.ekf_nis_gate
    P(6,6) = P(6,6) + 0.5*e(2)^2; P(5,5) = P(5,5) + 0.25*e(2)^2; w = 0;
end
S = H*P*H.' + Rm;
K = P*H.'/S;
x = x + K*e;
x(1) = min(max(x(1), 0), 1);
A = eye(6) - K*H;
P = A*P*A.' + K*Rm*K.';
soc = x(1); T_core = x(4); T_amb_est = x(6); innov = e(1); S_v = S(1,1);
P_soc = P(1,1); docv = ds(1);
% ---------------- time update ----------------
Tel = w*x(4) + (1-w)*Ts;
[v, ds, dT] = lut2(E, x(1), Tel);
R0 = v(2); R1 = v(3); t1 = max(v(4),1e-3); R2 = v(5); t2 = max(v(6),1e-3);
a1 = exp(-dt/t1); a2 = exp(-dt/t2);
if I >= 0, eta = 1; else, eta = E.eta_chg; end
dudt = interp1(E.soc_bp, E.dudt, min(max(x(1),0),1));
I0 = interp1(E.T_bp, E.I0_T, min(max(Tel,E.T_bp(1)),E.T_bp(end)));
eta_ct = 2*8.314462618*(Tel + 273.15)/96485.33212*asinh(I/(2*I0));
Q = I^2*R0 + I*eta_ct + I*(x(2) + x(3)) - I*(x(4) + 273.15)*dudt;
F = eye(6); F(2,2) = a1; F(3,3) = a2;
dT = dT*w;
da1 = a1*dt/t1^2*dT(4); da2 = a2*dt/t2^2*dT(6);
F(2,4) = (x(2) - R1*I)*da1 + (1 - a1)*I*dT(3);
F(3,4) = (x(3) - R2*I)*da2 + (1 - a2)*I*dT(5);
xn = zeros(6,1);
xn(1) = x(1) - eta*I*dt/(3600*E.Cn);
xn(2) = a1*x(2) + R1*(1 - a1)*I;
xn(3) = a2*x(3) + R2*(1 - a2)*I;
zt = E.Ad*[x(4); x(5)] + E.Bd*[Q; x(6)];
xn(4) = zt(1); xn(5) = zt(2); xn(6) = min(max(x(6), -40), 70);
dQ = [I^2*ds(2), I, I, I^2*dT(2) - I*dudt, 0, 0];
for r = 1:2
    F(3+r,:) = E.Bd(r,1)*dQ;
    F(3+r,4) = F(3+r,4) + E.Ad(r,1);
    F(3+r,5) = F(3+r,5) + E.Ad(r,2);
    F(3+r,6) = F(3+r,6) + E.Bd(r,2);
end
x = xn;
P = F*P*F.' + diag(E.ekf_Q);
w = 1 - E.ekf_trust_decay*(1 - w);
if I ~= 0
    ee = exp(-abs(I)*dt*E.hyst_gamma/(3600*E.Cn));
    h = ee*h - (1 - ee)*sign(I);
end
end

function [val, ds, dT] = lut2(E, soc, T)
% bilinear lookup of the 6 tables (OCV R0 R1 tau1 R2 tau2) and its partials
sb = E.soc_bp; tb = E.T_bp; ns = numel(sb); nt = numel(tb);
s = min(max(soc, sb(1)), sb(ns)); t = min(max(T, tb(1)), tb(nt));
i = 1; while i < ns-1 && s >= sb(i+1), i = i + 1; end
j = 1; while j < nt-1 && t >= tb(j+1), j = j + 1; end
u = (s - sb(i))/(sb(i+1) - sb(i)); q = (t - tb(j))/(tb(j+1) - tb(j));
val = zeros(6,1); ds = zeros(6,1); dT = zeros(6,1);
for k = 1:6
    f00 = E.tab(k,i,j); f10 = E.tab(k,i+1,j); f01 = E.tab(k,i,j+1); f11 = E.tab(k,i+1,j+1);
    val(k) = f00*(1-u)*(1-q) + f10*u*(1-q) + f01*(1-u)*q + f11*u*q;
    ds(k) = ((f10 - f00)*(1-q) + (f11 - f01)*q)/(sb(i+1) - sb(i));
    dT(k) = ((f01 - f00)*(1-u) + (f11 - f10)*u)/(tb(j+1) - tb(j));
end
end

function s0 = soc_from_v(E, V, T)
% rested-OCV inversion for the key-on initial SOC (linear interpolation
% on a 401-point grid of the OCV curve at the measured temperature)
cv = zeros(401,1); g = (0:400).'/400;
for k = 1:401
    [v, ~, ~] = lut2(E, g(k), T); cv(k) = v(1);
end
if V <= cv(1)
    s = 0;
elseif V >= cv(401)
    s = 1;
else
    k = 1; while cv(k+1) < V, k = k + 1; end
    s = g(k) + (V - cv(k))/(cv(k+1) - cv(k))*(g(k+1) - g(k));
end
s0 = min(max(s, 0.02), 0.98);
end

== matlab function EV_BMS_SOC_Estimation_System/9_SOC_Estimator_EKF_CNN_Fusion_1Hz/9b_1D_CNN_SOC_Estimator ==
  data: V input; soc_cnn output; I input; T input; valid output; d2 output; zmax output
function [soc_cnn, valid, d2, zmax] = CNN_SOC_Estimator(V, I, T)
%#codegen
% 1-D CNN SOC estimator, 1 Hz. Sliding 240 s window of 7 channels:
% v, i, t, i_ma (trailing 60 s mean), ah_cum (window-relative / Cn),
% dv (first difference), v_ir = v + i*R0_nom. Conv(16,k5)-BN-ReLU-Pool2,
% Conv(32,k5)-BN-ReLU-Pool2, Conv(64,k3)-BN-ReLU, GAP, Dense32-ReLU, Dense1-sigmoid.
N = coder.load('SOC_Estimator_Params.mat');   % weights: compile-time constants
persistent buf ibuf ah n vprev
if isempty(n)
    buf = zeros(240, 7); ibuf = zeros(60, 1); ah = zeros(240, 1); n = 0; vprev = V;
end
L = 240;
n = n + 1;
ibuf = [ibuf(2:end); I];
ima = sum(ibuf(max(1, 61 - n):60))/min(n, 60);
ahg = 0;
if n > 1, ahg = ah(end); end
ahg = ahg + I*1/3600;
ah = [ah(2:end); ahg];
if n == 1, dv = 0; else, dv = V - vprev; end
vprev = V;
buf = [buf(2:end,:); [V, I, T, ima, 0, dv, V + I*N.feat_R0]];
valid = double(n >= L);
soc_cnn = 0; d2 = 0; zmax = 0;
if n < L, return; end
X = buf;
X(:,5) = (ah - ah(1))/N.feat_Cn;
X = (X - repmat(N.nz_mean, L, 1)) ./ repmat(N.nz_std, L, 1);
% out-of-distribution statistics on the window-mean feature vector
f = mean(X, 1);
dd = f - N.ood_mu;
d2 = dd*N.ood_inv*dd.';
zmax = max(abs(dd ./ N.ood_sd));
% ---- network ----
a = conv_bn_relu(X, N.W1, N.b1, N.g1, N.be1, N.m1, N.v1, 5);
a = maxpool2(a);
a = conv_bn_relu(a, N.W2, N.b2, N.g2, N.be2, N.m2, N.v2, 5);
a = maxpool2(a);
a = conv_bn_relu(a, N.W3, N.b3, N.g3, N.be3, N.m3, N.v3, 3);
g = mean(a, 1);
h1 = max(g*N.W4 + N.b4, 0);
z = h1*N.W5 + N.b5;
soc_cnn = 1/(1 + exp(-min(max(z, -40), 40)));
end

function y = conv_bn_relu(x, W, b, gam, bet, mu, va, k)
% valid 1-D convolution, W is (k*Cin) x Cout with row index (j-1)*Cin + c
[Lx, C] = size(x); Lo = Lx - k + 1; Co = size(W, 2);
y = repmat(b, Lo, 1);
for j = 1:k
    y = y + x(j:j+Lo-1, :)*W((j-1)*C+1:j*C, :);
end
y = (y - repmat(mu, Lo, 1)) ./ repmat(sqrt(va + 1e-5), Lo, 1) .* repmat(gam, Lo, 1) + repmat(bet, Lo, 1);
y = max(y, 0);
end

function y = maxpool2(x)
[Lx, C] = size(x); Lt = floor(Lx/2);
y = zeros(Lt, C);
for r = 1:Lt
    y(r,:) = max(x(2*r-1,:), x(2*r,:));
end
end
